simulink model "model"  (R2024b)
settings: Solver=FixedStepDiscrete  StartTime=0.0  StopTime=30  FixedStep=0.1  RelTol=1e-3  EnableMultiTasking=on
libraries: stm32f4xxblockslib x6, stm32g4xxblockslib x2, stm32blockslib x2
(part 2 of 2)

== stateflow chart model/DomoticSystem ==
  state Active_State
    state Config_And_Operations [parallel]
      settings: executionOrder=1
      state Configuration
        state ERROR1
          en:
          uart_transmit_buffer = fromString2Bytes("\r\nInput too long: buffer overflow\r\nPress a key to continue...\r\n")
          uart_out_len = 100;
          ex:
          uart_out_len = 0;
        state Waiting
        state BlindsConfiguration
          state ManageInputBuffer1
            state waitForCompleteInput
              du:
              if uart_in_len == 1
              [input_buffer, new_bf_len, input_ovf] = updateInputBuffer(input_buffer, in_bf_len, uint8(uart_received_char));
              if new_bf_len ~= in_bf_len
              in_bf_len = new_bf_len
              uart_transmit_buffer = printInput(uart_received_char)
              uart_out_len = 1;
              end
              else
              uart_out_len = 0;
              end
              ex:
              uart_out_len = 0;
            (default) -> Active_State.Config_And_Operations.Configuration.BlindsConfiguration.ManageInputBuffer1.waitForCompleteInput
          state Validation
            en:
            [tmp_float_value, success] = asciiBufferToFloat(input_buffer, in_bf_len)
            config_err = ((mod(tmp_float_value, 20) ~= 0) || (tmp_float_value < 0 || tmp_float_value > 180))
          state InitCommunication2
            en:
            input_ovf = false;
            in_bf_len = uint32(0);
            uart_transmit_buffer = reset()
            input_buffer = uart_transmit_buffer(1:20)
            uart_transmit_buffer = cls();
            uart_out_len = 100;
          state PrintLightMenu
            en:
            uart_transmit_buffer = printBlindsMenu()
            uart_out_len = 100;
            ex:
            uart_out_len = 0;
          state SetAngle
            en:
            vblinds_angle = tmp_float_value
            uart_transmit_buffer = fromString2Bytes("\r\nBlinds Configured.\r\nPress a key to continue...\r\n")
            uart_out_len = 100;
            ex:
            uart_out_len = 0;
          state ERROR
            en:
            uart_transmit_buffer = fromString2Bytes("\r\nInvalid Input.\r\nPress a key to continue...\r\n")
            uart_out_len = 100;
            ex:
            uart_out_len = 0;
          state ERROR1
            en:
            uart_transmit_buffer = fromString2Bytes("\r\nInput too long: buffer overflow\r\nPress a key to continue...\r\n")
            uart_out_len = 100;
            ex:
            uart_out_len = 0;
          state Wait
          state Wait1
          state Wait2
          (default) -> Active_State.Config_And_Operations.Configuration.BlindsConfiguration.InitCommunication2
          Active_State.Config_And_Operations.Configuration.BlindsConfiguration.ManageInputBuffer1 -> Active_State.Config_And_Operations.Configuration.BlindsConfiguration.Validation [order 2] : [uart_received_char==EOS && uart_in_len == 1]
          Active_State.Config_And_Operations.Configuration.BlindsConfiguration.PrintLightMenu -> Active_State.Config_And_Operations.Configuration.BlindsConfiguration.ManageInputBuffer1
          Active_State.Config_And_Operations.Configuration.BlindsConfiguration.InitCommunication2 -> Active_State.Config_And_Operations.Configuration.BlindsConfiguration.PrintLightMenu
          Active_State.Config_And_Operations.Configuration.BlindsConfiguration.Validation -> Active_State.Config_And_Operations.Configuration.BlindsConfiguration.ERROR [order 1] : [config_err || ~success]
          Active_State.Config_And_Operations.Configuration.BlindsConfiguration.Validation -> Active_State.Config_And_Operations.Configuration.BlindsConfiguration.SetAngle [order 2]
          Active_State.Config_And_Operations.Configuration.BlindsConfiguration.ManageInputBuffer1 -> Active_State.Config_And_Operations.Configuration.BlindsConfiguration.ERROR1 [order 1] : [input_ovf]
          Active_State.Config_And_Operations.Configuration.BlindsConfiguration.ERROR -> Active_State.Config_And_Operations.Configuration.BlindsConfiguration.Wait
          Active_State.Config_And_Operations.Configuration.BlindsConfiguration.SetAngle -> Active_State.Config_And_Operations.Configuration.BlindsConfiguration.Wait2
          Active_State.Config_And_Operations.Configuration.BlindsConfiguration.ERROR1 -> Active_State.Config_And_Operations.Configuration.BlindsConfiguration.Wait1
          Active_State.Config_And_Operations.Configuration.BlindsConfiguration.Wait -> 466 : [uart_in_len == 1]
          Active_State.Config_And_Operations.Configuration.BlindsConfiguration.Wait1 -> 659 : [uart_in_len == 1]
          Active_State.Config_And_Operations.Configuration.BlindsConfiguration.Wait2 -> BlindsConfiguration : [uart_in_len == 1]{a_config_ended = true;
              | current_config_ended = true;}
        state PrintStatus
          en:
          uart_transmit_buffer = generateConfigurationStatus(isTempValid(temp), isAngleValid(vblinds_angle), isTimeValid(timer), isRelayValid(Relay))
          uart_out_len = 100;
          ex:
          uart_out_len = 0;
        state CheckOldValues
        state ManageInputBuffer
          state waitForCompleteInput
            du:
            if uart_in_len == 1
            [input_buffer, new_bf_len, input_ovf] = updateInputBuffer(input_buffer, in_bf_len, uint8(uart_received_char));
            if new_bf_len ~= in_bf_len
            in_bf_len = new_bf_len
            uart_transmit_buffer = printInput(uart_received_char)
            uart_out_len = 1;
            end
            else
            uart_out_len = 0;
            end
            ex:
            uart_out_len = 0;
          (default) -> Active_State.Config_And_Operations.Configuration.ManageInputBuffer.waitForCompleteInput
        state Validation
          en:
          [tmp_int_value, success] = asciiBufferToInt(input_buffer, in_bf_len)
          config_err = tmp_int_value >  3 || tmp_int_value < 1
        state LightConfiguration
          state InitCommunication3
            en:
            input_ovf = false;
            in_bf_len = uint32(0);
            uart_transmit_buffer = reset()
            input_buffer = uart_transmit_buffer(1:20)
            uart_transmit_buffer = cls();
            uart_out_len = 100;
          state ManageInputBuffer1
            state waitForCompleteInput
              du:
              if uart_in_len == 1
              [input_buffer, new_bf_len, input_ovf] = updateInputBuffer(input_buffer, in_bf_len, uint8(uart_received_char));
              if new_bf_len ~= in_bf_len
              in_bf_len = new_bf_len
              uart_transmit_buffer = printInput(uart_received_char)
              uart_out_len = 1;
              end
              else
              uart_out_len = 0;
              end
              ex:
              uart_out_len = 0;
            (default) -> Active_State.Config_And_Operations.Configuration.LightConfiguration.ManageInputBuffer1.waitForCompleteInput
          state InitCommunication2
            en:
            input_ovf = false;
            in_bf_len = uint32(0);
            uart_transmit_buffer = reset()
            input_buffer = uart_transmit_buffer(1:20)
            uart_transmit_buffer = cls();
            uart_out_len = 100;
          state PrintLightMenu
            en:
            uart_transmit_buffer = printLightMenu1()
            uart_out_len = 100;
            ex:
            uart_out_len = 0;
          state PrintLightTempMenu
            en:
            uart_transmit_buffer = printLightMenu2()
            uart_out_len = 100;
            ex:
            uart_out_len = 0;
          state Validation
            en:
            [tmp_int_value, success] = asciiBufferToInt(input_buffer, in_bf_len)
            config_err = tmp_int_value >  3 || tmp_int_value < 1
          state ManageInputBuffer2
            state waitForCompleteInput
              du:
              if uart_in_len == 1
              [input_buffer, new_bf_len, input_ovf] = updateInputBuffer(input_buffer, in_bf_len, uint8(uart_received_char));
              if new_bf_len ~= in_bf_len
              in_bf_len = new_bf_len
              uart_transmit_buffer = printInput(uart_received_char)
              uart_out_len = 1;
              end
              else
              uart_out_len = 0;
              end
              ex:
              uart_out_len = 0;
            (default) -> Active_State.Config_And_Operations.Configuration.LightConfiguration.ManageInputBuffer2.waitForCompleteInput
          state ERROR1
            en:
            uart_transmit_buffer = fromString2Bytes("\r\nInput too long: buffer overflow\r\nPress a key to continue...\r\n")
            uart_out_len = 100;
            ex:
            uart_out_len = 0;
          state ERROR
            en:
            uart_transmit_buffer = fromString2Bytes("\r\nInvalid Input.\r\nPress a key to continue...\r\n")
            uart_out_len = 100;
            ex:
            uart_out_len = 0;
          state Wait
          state SetLed
            en:
            Relay = boolean(tmp_int_value)
            uart_transmit_buffer = fromString2Bytes("\r\nRelay Configured.\r\nPress a key to continue...\r\n")
            uart_out_len = 100;
            ex:
            uart_out_len = 0;
          state Wait1
          state Validation1
            en:
            [tmp_float_value, success] = asciiBufferToFloat(input_buffer, in_bf_len)
            config_err = ~((tmp_float_value == 0) || (tmp_float_value >= 5 && tmp_float_value <= 30))
          state SetTime
            en:
            timer = tmp_float_value
            uart_transmit_buffer = fromString2Bytes("\r\nTemporization Configured.\r\nPress a key to continue...\r\n")
            uart_out_len = 100;
            ex:
            uart_out_len = 0;
          state Wait2
          Active_State.Config_And_Operations.Configuration.LightConfiguration.Validation -> InitCommunication3 [order 4] : [success && tmp_int_value==3]
          InitCommunication3 -> PrintLightTempMenu
          (default) -> Active_State.Config_And_Operations.Configuration.LightConfiguration.InitCommunication2
          Active_State.Config_And_Operations.Configuration.LightConfiguration.InitCommunication2 -> Active_State.Config_And_Operations.Configuration.LightConfiguration.PrintLightMenu
          Active_State.Config_And_Operations.Configuration.LightConfiguration.PrintLightMenu -> Active_State.Config_And_Operations.Configuration.LightConfiguration.ManageInputBuffer1
          Active_State.Config_And_Operations.Configuration.LightConfiguration.ManageInputBuffer1 -> Active_State.Config_And_Operations.Configuration.LightConfiguration.Validation [order 1] : [uart_received_char==EOS && uart_in_len == 1]
          Active_State.Config_And_Operations.Configuration.LightConfiguration.ManageInputBuffer1 -> Active_State.Config_And_Operations.Configuration.LightConfiguration.ERROR1 [order 2] : [input_ovf]
          PrintLightTempMenu -> ManageInputBuffer2
          Active_State.Config_And_Operations.Configuration.LightConfiguration.Validation -> SetLed [order 2] : [success && tmp_int_value==1]{tmp_int_value=int32(1)}
          Active_State.Config_And_Operations.Configuration.LightConfiguration.Validation -> SetLed [order 3] : [success && tmp_int_value==2]{tmp_int_value=int32(0)}
          Active_State.Config_And_Operations.Configuration.LightConfiguration.Validation -> Active_State.Config_And_Operations.Configuration.LightConfiguration.ERROR [order 1] : [config_err || ~success]
          ManageInputBuffer2 -> Active_State.Config_And_Operations.Configuration.LightConfiguration.ERROR1 [order 2] : [input_ovf]
          Active_State.Config_And_Operations.Configuration.LightConfiguration.ERROR1 -> Active_State.Config_And_Operations.Configuration.LightConfiguration.Wait
          ManageInputBuffer2 -> Validation1 [order 1] : [uart_received_char==EOS && uart_in_len == 1]
          Active_State.Config_And_Operations.Configuration.LightConfiguration.ERROR -> Active_State.Config_And_Operations.Configuration.LightConfiguration.Wait1
          Validation1 -> Active_State.Config_And_Operations.Configuration.LightConfiguration.ERROR [order 1] : [config_err || ~success]
          Active_State.Config_And_Operations.Configuration.LightConfiguration.Wait -> 593 : [uart_in_len == 1]
          Active_State.Config_And_Operations.Configuration.LightConfiguration.Wait1 -> 442 : [uart_in_len == 1]
          SetLed -> Active_State.Config_And_Operations.Configuration.LightConfiguration.Wait2
          Validation1 -> SetTime [order 2] : [success]
          SetTime -> Active_State.Config_And_Operations.Configuration.LightConfiguration.Wait2
          Active_State.Config_And_Operations.Configuration.LightConfiguration.Wait2 -> LightConfiguration : [uart_in_len == 1]{a_config_ended = true;
              | current_config_ended = true;}
        state PrintMenu
          en:
          uart_transmit_buffer=printMenu()
          uart_out_len = 100;
          ex:
          uart_out_len = 0;
        state InitCommunication1
          en:
          input_ovf = false;
          in_bf_len = uint32(0);
          uart_transmit_buffer = reset()
          input_buffer = uart_transmit_buffer(1:20)
          uart_transmit_buffer = cls();
          uart_out_len = 100;
        state init
          en:
          if ~a_config_ended
          a_config_ended  = false
          end
        state feedback
          en:
          uart_transmit_buffer = fromString2Bytes("\r\nInvalid input.\r\nPress a key to continue...\r\n")
          uart_out_len = 100;
          ex:
          uart_out_len = 0;
        state Wait
        state HeatConfiguration
          state ManageInputBuffer1
            state waitForCompleteInput
              du:
              if uart_in_len == 1
              [input_buffer, new_bf_len, input_ovf] = updateInputBuffer(input_buffer, in_bf_len, uint8(uart_received_char));
              if new_bf_len ~= in_bf_len
              in_bf_len = new_bf_len
              uart_transmit_buffer = printInput(uart_received_char)
              uart_out_len = 1;
              end
              else
              uart_out_len = 0;
              end
              ex:
              uart_out_len = 0;
            (default) -> Active_State.Config_And_Operations.Configuration.HeatConfiguration.ManageInputBuffer1.waitForCompleteInput
          state Validation
            en:
            [tmp_float_value, success] = asciiBufferToFloat(input_buffer, in_bf_len)
            config_err = ((abs(mod(tmp_float_value,1)) > 1e-10) || (tmp_float_value < 16 || tmp_float_value > 30))
          state InitCommunication2
            en:
            input_ovf = false;
            in_bf_len = uint32(0);
            uart_transmit_buffer = reset()
            input_buffer = uart_transmit_buffer(1:20)
            uart_transmit_buffer = cls();
            uart_out_len = 100;
          state PrintLightMenu
            en:
            uart_transmit_buffer = printBlindsMenu()
            uart_out_len = 100;
            ex:
            uart_out_len = 0;
          state ERROR
            en:
            uart_transmit_buffer = fromString2Bytes("\r\nInvalid Input.\r\nPress a key to continue...\r\n")
            uart_out_len = 100;
            ex:
            uart_out_len = 0;
          state SetTemp
            en:
            temp = tmp_float_value
            uart_transmit_buffer = fromString2Bytes("\r\nTemperature Configured.\r\nPress a key to continue...\r\n")
            uart_out_len = 100;
            ex:
            uart_out_len = 0;
          state ERROR1
            en:
            uart_transmit_buffer = fromString2Bytes("\r\nInput too long: buffer overflow\r\nPress a key to continue...\r\n")
            uart_out_len = 100;
            ex:
            uart_out_len = 0;
          state Wait1
          state Wait
          state Wait2
          (default) -> Active_State.Config_And_Operations.Configuration.HeatConfiguration.InitCommunication2
          Active_State.Config_And_Operations.Configuration.HeatConfiguration.ManageInputBuffer1 -> Active_State.Config_And_Operations.Configuration.HeatConfiguration.Validation [order 2] : [uart_received_char==EOS && uart_in_len == 1]
          Active_State.Config_And_Operations.Configuration.HeatConfiguration.PrintLightMenu -> Active_State.Config_And_Operations.Configuration.HeatConfiguration.ManageInputBuffer1
          Active_State.Config_And_Operations.Configuration.HeatConfiguration.InitCommunication2 -> Active_State.Config_And_Operations.Configuration.HeatConfiguration.PrintLightMenu
          Active_State.Config_And_Operations.Configuration.HeatConfiguration.Validation -> Active_State.Config_And_Operations.Configuration.HeatConfiguration.ERROR [order 1] : [config_err || ~success]
          Active_State.Config_And_Operations.Configuration.HeatConfiguration.Validation -> SetTemp [order 2]
          Active_State.Config_And_Operations.Configuration.HeatConfiguration.ManageInputBuffer1 -> Active_State.Config_And_Operations.Configuration.HeatConfiguration.ERROR1 [order 1] : [input_ovf]
          Active_State.Config_And_Operations.Configuration.HeatConfiguration.ERROR1 -> Active_State.Config_And_Operations.Configuration.HeatConfiguration.Wait
          Active_State.Config_And_Operations.Configuration.HeatConfiguration.ERROR -> Active_State.Config_And_Operations.Configuration.HeatConfiguration.Wait1
          SetTemp -> Active_State.Config_And_Operations.Configuration.HeatConfiguration.Wait2
          Active_State.Config_And_Operations.Configuration.HeatConfiguration.Wait -> 601 : [uart_in_len == 1]
          Active_State.Config_And_Operations.Configuration.HeatConfiguration.Wait1 -> 482 : [uart_in_len == 1]
          Active_State.Config_And_Operations.Configuration.HeatConfiguration.Wait2 -> HeatConfiguration : [uart_in_len == 1]{a_config_ended = true;
              | current_config_ended = true;}
        CheckOldValues -> init
        Waiting -> CheckOldValues : [uart_in_len == 1]
        Active_State.Config_And_Operations.Configuration.ERROR1 -> Waiting
        ManageInputBuffer -> Active_State.Config_And_Operations.Configuration.ERROR1 [order 2] : [input_ovf]
        BlindsConfiguration -> Configuration : [current_config_ended]
        Active_State.Config_And_Operations.Configuration.Validation -> BlindsConfiguration [order 1] : [tmp_int_value == 1]{current_config_ended=false}
        660 -> CheckOldValues
        473 -> CheckOldValues
        602 -> CheckOldValues
        596 -> CheckOldValues
        480 -> CheckOldValues
        443 -> CheckOldValues
        PrintStatus -> PrintMenu
        PrintMenu -> ManageInputBuffer
        Active_State.Config_And_Operations.Configuration.Validation -> LightConfiguration [order 3] : [tmp_int_value == 2]{current_config_ended=false}
        ManageInputBuffer -> Active_State.Config_And_Operations.Configuration.Validation [order 1] : [uart_received_char==EOS && uart_in_len == 1]
        LightConfiguration -> Configuration : [current_config_ended]
        Active_State.Config_And_Operations.Configuration.Validation -> HeatConfiguration [order 4] : [tmp_int_value == 3]{current_config_ended=false}
        InitCommunication1 -> PrintStatus
        init -> InitCommunication1
        Active_State.Config_And_Operations.Configuration.Validation -> feedback [order 2] : [~success || config_err]
        Active_State.Config_And_Operations.Configuration.Wait -> InitCommunication1 : [uart_in_len == 1]
        (default) -> init
        feedback -> Active_State.Config_And_Operations.Configuration.Wait
        HeatConfiguration -> Configuration : [current_config_ended]
      state WaitForRelease1
      state Operational
        state HeatingManagement [parallel]
          settings: executionOrder=4
          state range_1
            en:
            Heating_R = 255;
            Heating_G = 255;
            Heating_B = 0;
          state range_2
            en:
            Heating_R = 128;
            Heating_G = 255;
            Heating_B = 128;
          state range_4
            en:
            Heating_R = 0;
            Heating_G = 128;
            Heating_B = 255;
          state range_3
            en:
            Heating_R = 0;
            Heating_G = 0;
            Heating_B = 255;
          state range_5
            en:
            Heating_R = 0;
            Heating_G = 255;
            Heating_B = 255;
          (default) -> (junction 715)
          range_5 -> (junction 715) : [temp>30]
          (junction 715) -> range_1 [order 1] : [temp>=16 && temp<=18]
          (junction 715) -> range_5 [order 5] : [temp>= 28 && temp<=30]
          range_1 -> (junction 715) : [temp>18]
          range_4 -> (junction 715) : [temp>27]
          (junction 715) -> range_2 [order 2] : [temp>=19 && temp<=21]
          (junction 715) -> range_4 [order 4] : [temp>= 25 && temp<=27]
          range_2 -> (junction 715) : [temp>21]
          range_3 -> (junction 715) : [temp>24]
          (junction 715) -> range_3 [order 3] : [temp>=22 && temp<=24]
        state LightManagement [parallel]
          settings: executionOrder=2
          state Relay
            state Operation
              state OFF
                state WaitForButtonPressing
                state Debounce
                state Turn_off
                  en:
                  Relay=OFF;
                Active_State.Config_And_Operations.Operational.LightManagement.Relay.Operation.OFF.Debounce -> Active_State.Config_And_Operations.Operational.LightManagement.Relay.Operation.OFF.WaitForButtonPressing : after(debounce, sec)
                Turn_off -> Active_State.Config_And_Operations.Operational.LightManagement.Relay.Operation.OFF.Debounce : [button_light_pressed==OFF]
                (default) -> Turn_off
              state ON
                state Turn_ON
                  en:
                  Relay=ON
                state Debounce
                state WaitForButtonPressing
                (default) -> Turn_ON
                Turn_ON -> Active_State.Config_And_Operations.Operational.LightManagement.Relay.Operation.ON.Debounce : [button_light_pressed==OFF]
                Active_State.Config_And_Operations.Operational.LightManagement.Relay.Operation.ON.Debounce -> Active_State.Config_And_Operations.Operational.LightManagement.Relay.Operation.ON.WaitForButtonPressing : after(debounce, sec)
              (default) -> (junction 643)
              (junction 643) -> Active_State.Config_And_Operations.Operational.LightManagement.Relay.Operation.ON [order 2] : [Relay==ON]
              (junction 643) -> Active_State.Config_And_Operations.Operational.LightManagement.Relay.Operation.OFF [order 1] : [Relay==OFF]
              Active_State.Config_And_Operations.Operational.LightManagement.Relay.Operation.OFF.WaitForButtonPressing -> Active_State.Config_And_Operations.Operational.LightManagement.Relay.Operation.ON : [button_light_pressed==ON]
              Active_State.Config_And_Operations.Operational.LightManagement.Relay.Operation.ON.WaitForButtonPressing -> Turn_off : [button_light_pressed==ON]
            state Debounce
            state Temp
              state GoToRelay [parallel]
                settings: executionOrder=1
                state WaitForPressing
                (default) -> WaitForPressing
              state EllapsedTime [parallel]
                settings: executionOrder=2
                state Wait
                  en:
                  Relay=ON;
                (default) -> Active_State.Config_And_Operations.Operational.LightManagement.Relay.Temp.EllapsedTime.Wait
            state WaitForRelease
            state Debounce1
            (default) -> Operation
            Active_State.Config_And_Operations.Operational.LightManagement.Relay.Temp.EllapsedTime.Wait -> Operation : [after(timer, sec)]{Relay=OFF}
            Active_State.Config_And_Operations.Operational.LightManagement.Relay.Debounce -> Operation : after(debounce, sec){Relay=OFF}
            Operation -> Active_State.Config_And_Operations.Operational.LightManagement.Relay.WaitForRelease : [button_temp_pressed==ON && uint32(timer) ~= 0]
            WaitForPressing -> Active_State.Config_And_Operations.Operational.LightManagement.Relay.Debounce : [button_light_pressed==ON && button_temp_pressed==OFF]
            Active_State.Config_And_Operations.Operational.LightManagement.Relay.WaitForRelease -> Active_State.Config_And_Operations.Operational.LightManagement.Relay.Debounce1 : [button_temp_pressed==OFF]
            Active_State.Config_And_Operations.Operational.LightManagement.Relay.Debounce1 -> Temp : [after(debounce, sec)]
          (default) -> Relay
        state NotifyUART [parallel]
          settings: executionOrder=3
          state Invia
            en:
            uart_transmit_buffer = messageForUART(Relay,vblinds_angle,temp,timer)
            uart_out_len = 100
            ex:
            uart_out_len = 0
          state Wait
          (default) -> Invia
          Invia -> Active_State.Config_And_Operations.Operational.NotifyUART.Wait
          Active_State.Config_And_Operations.Operational.NotifyUART.Wait -> Invia : after(10, sec)
        state VBlindsManagement [parallel]
          settings: executionOrder=1
          state SetAngle
            du:
            servo_pwm_out = 5.0 + (vblinds_angle / 180.0) * 20.0;
          (default) -> Active_State.Config_And_Operations.Operational.VBlindsManagement.SetAngle
      state Debounce3
      state WaitForRelease
      state Debounce2
      (junction 674) -> Configuration [order 1] : [first_config]
      (default) -> (junction 674)
      (junction 674) -> Operational [order 2]
      Configuration -> WaitForRelease1 : [a_config_ended  == true && button_config_pressed==ON && isTempValid(temp) && isAngleValid(vblinds_angle) && isTimeValid(timer) && isRelayValid(Relay)]{first_config=false}
      WaitForRelease1 -> Debounce3 : [button_temp_pressed==OFF]
      Debounce3 -> Operational : after(debounce, sec)
      Active_State.Config_And_Operations.WaitForRelease -> Debounce2 : [button_temp_pressed==OFF]
      Debounce2 -> Configuration : after(debounce, sec){a_config_ended = false}
      Operational -> Active_State.Config_And_Operations.WaitForRelease : [button_config_pressed==ON]
    state BlinkingManagement [parallel]
      settings: executionOrder=2
      state ON
        en:
        Blinking=ON
      state OFF
        en:
        Blinking=OFF
      (default) -> Active_State.BlinkingManagement.ON
      Active_State.BlinkingManagement.OFF -> Active_State.BlinkingManagement.ON : after(1/(2*blinking_hz), sec)
      Active_State.BlinkingManagement.ON -> Active_State.BlinkingManagement.OFF : after(1/(2*blinking_hz), sec)
  state PopValues
    en:
    tmp_float_value = tmp_float_value_Old_Session;
    Relay = Relay_Old_Session;
    Heating_R = Heating_R_Old_Session ;
    Heating_G = Heating_G_Old_Session;
    Heating_B = Heating_B_Old_Session;
    servo_pwm_out = servo_pwm_out_Old_Session;
    vblinds_angle = vblinds_angle_Old_Session;
  state Debounce
    en:
    uart_out_len = 0
  state WaitForRelese
    en:
    uart_transmit_buffer = cls()
    uart_out_len = 100
    ex:
    uart_out_len = 0
  state OFF_STATE
    en:
    % Push Values
    Relay_Old_Session = Relay;
    Heating_R_Old_Session = Heating_R;
    Heating_G_Old_Session = Heating_G;
    Heating_B_Old_Session = Heating_B;
    servo_pwm_out_Old_Session = servo_pwm_out;
    vblinds_angle_Old_Session = vblinds_angle;
    tmp_float_value_Old_Session = tmp_float_value
    % Tutto Spento
    Blinking=OFF;
    Relay = OFF;
    Heating_R = 255;
    Heating_G = 255;
    Heating_B = 255;
    servo_pwm_out = 5.0;
    vblinds_angle = 0.0;
    %Print
    uart_transmit_buffer = fromString2Bytes(sprintf('\033[0;0H\033[2J') + "[Inactive State]");
    uart_out_len = 100;
    ex:
    uart_out_len = 0;
  state Wait
  state WaitForRelese1
    en:
    uart_transmit_buffer = cls()
    uart_out_len = 100
    ex:
    uart_out_len = 0
  state Debounce1
    en:
    uart_out_len = 0
  PopValues -> Active_State
  Debounce -> PopValues : after(debounce, sec)
  WaitForRelese -> Debounce : [power_button_pressed==OFF]
  (default) -> OFF_STATE
  Wait -> WaitForRelese : [power_button_pressed==ON]
  OFF_STATE -> Wait
  Active_State -> WaitForRelese1 : [power_button_pressed==ON]
  WaitForRelese1 -> Debounce1 : [power_button_pressed==OFF]
  Debounce1 -> OFF_STATE : after(debounce, sec)
  data: buffer function_output uint8 size=100; buffer function_output uint8 size=100; buffer function_output uint8 size=100; buffer function_output uint8 size=100; isTempValid function_input; isAngleValid function_input; isTimeValid function_input; isRelayValid function_input; msg function_output; msg_len function_output; input_buffer function_input uint8 size=20; length function_input uint32 size=1; inputChar function_input uint8 size=1; new_input_buffer function_output uint8 size=20; newLength function_output uint32 size=1; overflow function_output boolean size=1; buffer function_output uint8 size=100; buffer function_input; length function_input; value function_output; success function_output; buffer function_output uint8 size=100; input function_input uint8 size=1; buffer function_input; length function_input; value function_output; success function_output; input_buffer function_input; formatted_buffer function_output; out_len function_output; buffer function_output uint8 size=100; angle function_input; validation function_output; temp function_input; validation function_output; relay function_input boolean size=1; validation function_output boolean size=1; str function_input; msg function_output; time function_input; validation function_output; buffer function_output uint8 size=100; relay function_input boolean size=1; angle function_input; temperature function_input double size=1; temporization function_input double size=1; msg function_output uint8 size=100; msg_len function_output uint32 size=1; ON constant boolean =1; OFF constant boolean =0; Relay output boolean size=1 =0; button_light_pressed input boolean size=1; button_temp_pressed input boolean size=1; debounce local double size=1 =0.05; timer local double size=1 =-1; blinking_hz local double size=1 =2; Blinking output; Heating_B output uint8 size=1 =255; Heating_R output uint8 size=1 =255; Heating_G output uint8 size=1 =255; button_config_pressed input boolean size=1; uart_transmit_buffer output uint8 size=100; uart_out_len output uint8 size=1; uart_received_char input uint8 size=1; uart_in_len input uint32 size=1; input_buffer local uint8 size=20; in_bf_len local uint32 size=1; EOS constant uint8 =13; tmp_int_value local int32 size=1 =0; success local boolean size=1 =0; tmp_float_value local double size=1 =-1.0; config_err local boolean size=1 =0; new_bf_len local uint32 size=1; vblinds_angle local double size=1 =-1; temp local double size=1 =-1; input_ovf local boolean size=1; current_config_ended local; a_config_ended local boolean size=1 =0; power_button_pressed input boolean size=1; servo_pwm_out output double size=1; first_config local boolean size=1 =true; Heating_B_Old_Session local; Heating_G_Old_Session local; Heating_R_Old_Session local; Relay_Old_Session local; servo_pwm_out_Old_Session local; vblinds_angle_Old_Session local; tmp_float_value_Old_Session local
  function buffer = printBlindsMenu:
    | function buffer = printBlindsMenu() %#codegen
    | % Restituisce un vettore uint8 (MAX_LEN × 1) con il menu testuale.
    | 
    | MAX_LEN = 100;
    | buffer  = zeros(MAX_LEN, 1, 'uint8');
    | idx     = int32(1);
    | 
    | % Char-matrix a lunghezza fissa (ogni riga 25 caratteri in questo esempio)
    | menu = [ ...
    |     'Blinds Menu:                                          '; ... % 
    |     'Insert the angle in degree with a resolution of 20    '; ... % 
    |     'inclusive range: 0-180                                '
    |     'Insert:                                               '  ... %
    | ];
    | 
    | nLines  = size(menu, 1);
    | nCols   = size(menu, 2);            % lunghezza fissa di ogni riga
    | 
    | for i = 1:nLines
    |     % Trova l’ultima colonna non-spazio della riga i
    |     last = int32(0);
    |     for c = nCols:-1:1
    |         if menu(i, c) ~= ' '
    |             last = int32(c);
    |             break;
    |         end
    |     end
    | 
    |     % Copia i caratteri utili
    |     for k = int32(1):last
    |         buffer(idx) = uint8(menu(i, k));
    |         idx = idx + 1;
    |     end
    |     
    |     % tmp = buffer(1:199)
    |     % Aggiunge newline '\n'
    |     buffer(idx) = uint8(10);
    |     idx = idx + 1;
    |     buffer(idx) = uint8(13);
    |     idx = idx + 1;
    | end
    | end
  function buffer = printLightMenu1:
    | function buffer = printLightMenu1() %#codegen
    | % Restituisce un vettore uint8 (MAX_LEN × 1) con il menu testuale.
    | 
    | MAX_LEN = 100;
    | buffer  = zeros(MAX_LEN, 1, 'uint8');
    | idx     = int32(1);
    | 
    | % Char-matrix a lunghezza fissa (ogni riga 25 caratteri in questo esempio)
    | menu = [ ...
    |     'Light Menu:      '; ... % 
    |     '1 - Turn On      '; ... % 
    |     '2 - Turn Off     '; ... % 
    |     '3 - Temporization'; ... % 
    |     'Insert:          '  ... %
    | ];
    | 
    | nLines  = size(menu, 1);
    | nCols   = size(menu, 2);            % lunghezza fissa di ogni riga
    | 
    | for i = 1:nLines
    |     % Trova l’ultima colonna non-spazio della riga i
    |     last = int32(0);
    |     for c = nCols:-1:1
    |         if menu(i, c) ~= ' '
    |             last = int32(c);
    |             break;
    |         end
    |     end
    | 
    |     % Copia i caratteri utili
    |     for k = int32(1):last
    |         buffer(idx) = uint8(menu(i, k));
    |         idx = idx + 1;
    |     end
    |     
    |     % tmp = buffer(1:199)
    |     % Aggiunge newline '\n'
    |     buffer(idx) = uint8(10);
    |     idx = idx + 1;
    |     buffer(idx) = uint8(13);
    |     idx = idx + 1;
    | end
    | end
  function buffer = printLightMenu2:
    | function buffer = printLightMenu2() %#codegen
    | % Restituisce un vettore uint8 (MAX_LEN × 1) con il menu testuale.
    | 
    | MAX_LEN = 100;
    | buffer  = zeros(MAX_LEN, 1, 'uint8');
    | idx     = int32(1);
    | 
    | % Char-matrix a lunghezza fissa (ogni riga 25 caratteri in questo esempio)
    | menu = [ ...
    |     'Temporization Menu:                                                    '; ... % 
    |     'You can either enter 0 or a value between the inclusive range 5...30   '; ... % 
    |     'Insert:                                                                '  ... %
    | ];
    | 
    | nLines  = size(menu, 1);
    | nCols   = size(menu, 2);            % lunghezza fissa di ogni riga
    | 
    | for i = 1:nLines
    |     % Trova l’ultima colonna non-spazio della riga i
    |     last = int32(0);
    |     for c = nCols:-1:1
    |         if menu(i, c) ~= ' '
    |             last = int32(c);
    |             break;
    |         end
    |     end
    | 
    |     % Copia i caratteri utili
    |     for k = int32(1):last
    |         buffer(idx) = uint8(menu(i, k));
    |         idx = idx + 1;
    |     end
    |     
    |     % tmp = buffer(1:199)
    |     % Aggiunge newline '\n'
    |     buffer(idx) = uint8(10);
    |     idx = idx + 1;
    |     buffer(idx) = uint8(13);
    |     idx = idx + 1;
    | end
    | end
  function buffer = printBlindsMenu:
    | function buffer = printBlindsMenu() %#codegen
    | % Restituisce un vettore uint8 (MAX_LEN × 1) con il menu testuale.
    | 
    | MAX_LEN = 100;
    | buffer  = zeros(MAX_LEN, 1, 'uint8');
    | idx     = int32(1);
    | 
    | % Char-matrix a lunghezza fissa (ogni riga 25 caratteri in questo esempio)
    | menu = [ ...
    |     'Heating Menu:                    '; ... % 
    |     'Insert the temperature in celsius'; ... %
    |     'Resolution: 1 C                  '
    |     'Inclusive range: 16-30           '
    |     'Insert:                          '  ... %
    | ];
    | 
    | nLines  = size(menu, 1);
    | nCols   = size(menu, 2);            % lunghezza fissa di ogni riga
    | 
    | for i = 1:nLines
    |     % Trova l’ultima colonna non-spazio della riga i
    |     last = int32(0);
    |     for c = nCols:-1:1
    |         if menu(i, c) ~= ' '
    |             last = int32(c);
    |             break;
    |         end
    |     end
    | 
    |     % Copia i caratteri utili
    |     for k = int32(1):last
    |         buffer(idx) = uint8(menu(i, k));
    |         idx = idx + 1;
    |     end
    |     
    |     % tmp = buffer(1:199)
    |     % Aggiunge newline '\n'
    |     buffer(idx) = uint8(10);
    |     idx = idx + 1;
    |     buffer(idx) = uint8(13);
    |     idx = idx + 1;
    | end
    | end
  function [msg, msg_len] = generateConfigurationStatus(isTempValid, isAngleValid, isTimeValid, isRelayValid):
    | function [msg, msg_len] = generateConfigurationStatus(isTempValid, isAngleValid, isTimeValid, isRelayValid)
    | %#codegen
    | % Questa funzione genera la linea di stato per il menu di configurazione.
    | % Es: 
    | % [Configuration]
    | % Tempe: x Angle: o Timer: x Relay: o
    | % È progettata per essere efficiente e compatibile con Stateflow (#codegen).
    | 
    |     % Buffer per contenere il messaggio. 128 è più che sufficiente.
    |     MAX_LEN = 100;
    |     persistent msg_buffer
    |     if isempty(msg_buffer)
    |         msg_buffer = zeros(MAX_LEN, 1, 'uint8');
    |     end
    |     
    |     % Pulisce il buffer per ogni nuova chiamata.
    |     msg_buffer(:) = 0;
    |     
    |     % Usa uint32 per il contatore per compatibilità con l'output msg_len.
    |     idx = uint32(1);
    |     
    |     % --- Costruzione del Messaggio ---
    | 
    |     % Riga 1: Titolo e a capo
    |     [msg_buffer, idx] = write_string('[Configuration]', msg_buffer, idx);
    |     msg_buffer(idx) = uint8(10); % Newline (LF, \n)
    |     idx = idx + 1;
    |     msg_buffer(idx) = uint8(13); % Carriage Return (LF, \r)
    |     idx = idx + 1;
    |     
    |     % Riga 2: Stato delle variabili
    |     
    |     % Temperatura
    |     [msg_buffer, idx] = write_string('Tempe: ', msg_buffer, idx);
    |     if isTempValid
    |         msg_buffer(idx) = uint8('o');
    |     else
    |         msg_buffer(idx) = uint8('x');
    |     end
    |     idx = idx + 1;
    |     
    |     % Angolo (con spazio iniziale per separare)
    |     [msg_buffer, idx] = write_string(' Angle: ', msg_buffer, idx);
    |     if isAngleValid
    |         msg_buffer(idx) = uint8('o');
    |     else
    |         msg_buffer(idx) = uint8('x');
    |     end
    |     idx = idx + 1;
    | 
    |     % Timer (con spazio iniziale)
    |     [msg_buffer, idx] = write_string(' Timer: ', msg_buffer, idx);
    |     if isTimeValid
    |         msg_buffer(idx) = uint8('o');
    |     else
    |         msg_buffer(idx) = uint8('x');
    |     end
    |     idx = idx + 1;
    | 
    |     % Relay (con spazio iniziale)
    |     [msg_buffer, idx] = write_string(' Relay: ', msg_buffer, idx);
    |     if isRelayValid
    |         msg_buffer(idx) = uint8('o');
    |     else
    |         msg_buffer(idx) = uint8('x');
    |     end
    |     idx = idx + 1;
    | 
    |     % --- Terminazione del messaggio completo (LF + CR) ---
    |     msg_buffer(idx) = uint8(10); % LF (\n)
    |     idx = idx + 1;
    |     msg_buffer(idx) = uint8(13); % CR (\r)
    |     idx = idx + 1;
    |     
    |     % Imposta i valori di output
    |     msg_len = idx - 1;
    |     msg = msg_buffer;
    | end
    | 
    | 
    | % --- FUNZIONE LOCALE DI SUPPORTO ---
    | 
    | function [msg, idx_out] = write_string(str, msg, idx_in)
    | %#codegen
    | % Scrive una stringa di caratteri nel buffer in modo efficiente.
    |     str_as_uint8 = uint8(str);
    |     len = uint32(numel(str_as_uint8)); % Usa uint32 per coerenza
    |     for k = 1:len
    |         % L'indice del buffer deve essere un intero, quindi usiamo (idx_in + k - 1)
    |         % e Coder gestisce la conversione da uint32 a double per l'indicizzazione.
    |         msg(idx_in + (k - 1)) = str_as_uint8(k);
    |     end
    |     idx_out = idx_in + len;
    | end
  function [new_input_buffer, newLength, overflow] = updateInputBuffer(input_buffer, length, inputChar):
    | function [new_input_buffer, newLength, overflow] = updateInputBuffer(input_buffer, length, inputChar)
    | %#codegen
    | % Aggiorna un buffer di input con un nuovo carattere.
    | % Gestisce cifre, backspace e invio (che termina la stringa con '\0').
    | 
    | MAX_LEN = 20;
    | overflow = false;
    | new_input_buffer = input_buffer;
    | newLength = length;
    | inputChar = uint8((inputChar));
    | 
    | % Se il carattere è una cifra '0'-'9'
    | if inputChar >= uint8(('0')) && inputChar <= uint8(('9'))
    |     if newLength < MAX_LEN
    |         new_input_buffer(newLength + 1) = inputChar;
    |         newLength = newLength + 1;
    |     else
    |         overflow = true;
    |     end
    | 
    | % Se il carattere è BACKSPACE (ASCII 8) o DELETE (ASCII 127)
    | elseif inputChar == 8 || inputChar == 127
    |     if newLength > 0
    |         % Rimuove l'ultimo carattere (non è necessario azzerarlo se
    |         % la lunghezza è gestita correttamente, ma è una buona pratica)
    |         new_input_buffer(newLength) = uint8((0)); 
    |         newLength = newLength - 1;
    |     end
    | 
    | % Se il carattere è INVIO (ENTER, ASCII 13)
    | elseif inputChar == 13
    |     % Aggiunge il terminatore di stringa C-style '\0'
    |     if newLength < MAX_LEN
    |         new_input_buffer(newLength + 1) = uint8((0));
    |         % Non è necessario incrementare newLength per il terminatore,
    |         % perché la lunghezza utile non lo include. Ma se lo fai,
    |         % assicurati di essere coerente. Lasciamolo così per ora.
    |     else
    |         overflow = true;
    |     end
    |     % La logica che riempie il resto del buffer con zeri è superflua
    |     % se la funzione di conversione si ferma al primo zero, ma la manteniamo
    |     % per sicurezza e pulizia del buffer.
    |     for k = newLength+2:MAX_LEN
    |         new_input_buffer(k) = uint8((0));
    |     end
    | elseif inputChar == uint8(('.'))
    |     already_used = false;
    |     for i=1:newLength
    |         if new_input_buffer(i) == uint8(('.'))
    |             already_used = true;
    |             break
    |         end
    |     end
    |     if already_used == false
    |         if newLength + 1 < MAX_LEN
    |             new_input_buffer(newLength + 1) = inputChar;
    |             newLength = newLength + 1;
    |         else
    |             overflow = true;
    |         end
    |     end
    | else
    |     % Ignora esplicitamente tutti gli altri caratteri.
    |     % Se 'inputChar' è un carattere non gestito (es. 'a', '!', o un codice
    |     % di escape inviato dal tasto CANC), la funzione non farà nulla,
    |     % restituendo il buffer e la lunghezza inalterati.
    |     % Questo risolve il tuo problema.
    | end
    | 
    | 
    | 
    | return
    | end
  function buffer = printMenu:
    | function buffer = printMenu() %#codegen
    | % Restituisce un vettore uint8 (MAX_LEN × 1) con il menu testuale.
    | 
    | MAX_LEN = 100;
    | buffer  = zeros(MAX_LEN, 1, 'uint8');
    | idx     = int32(1);
    | 
    | % Char-matrix a lunghezza fissa (ogni riga 25 caratteri in questo esempio)
    | menu = [ ...
    |     'Config Menu:            '; ... % 
    |     '1 - Blinds Configuration'; ... % 
    |     '2 - Light Configuration '; ... % 
    |     '3 - Heat Configuration  '; ... % 
    |     'Insert:                 '  ... %
    | ];
    | 
    | nLines  = size(menu, 1);
    | nCols   = size(menu, 2);            % lunghezza fissa di ogni riga
    | 
    | for i = 1:nLines
    |     % Trova l’ultima colonna non-spazio della riga i
    |     last = int32(0);
    |     for c = nCols:-1:1
    |         if menu(i, c) ~= ' '
    |             last = int32(c);
    |             break;
    |         end
    |     end
    | 
    |     % Copia i caratteri utili
    |     for k = int32(1):last
    |         buffer(idx) = uint8(menu(i, k));
    |         idx = idx + 1;
    |     end
    |     
    |     % tmp = buffer(1:199)
    |     % Aggiunge newline '\n'
    |     buffer(idx) = uint8(10);
    |     idx = idx + 1;
    |     buffer(idx) = uint8(13);
    |     idx = idx + 1;
    | end
    | end
  function [value, success] = asciiBufferToInt(buffer, length):
    | function [value, success] = asciiBufferToInt(buffer, length)
    | %#codegen
    | % Converte un buffer di caratteri ASCII in un intero a 32 bit.
    | % Si ferma al primo carattere nullo '\0' o alla fine della 'length' data.
    | 
    | value = int32(0);
    | success = true;
    | 
    | if length == 0
    |     success = false;
    |     return;
    | end
    | 
    | sign = int32(1);
    | startIdx = 1;
    | 
    | % Gestisce il segno
    | if buffer(1) == uint8('-')
    |     sign = int32(-1);
    |     startIdx = 2;
    | elseif buffer(1) == uint8('+')
    |     startIdx = 2;
    | end
    | 
    | % Itera sui caratteri fino alla lunghezza specificata
    | for i = startIdx:length
    |     c = buffer(i);
    |     
    |     % Se incontra il terminatore di stringa, la conversione è finita e ha successo
    |     if c == 0
    |         break;
    |     end
    |     
    |     % Se il carattere non è una cifra, la conversione fallisce
    |     if c < '0' || c > '9'
    |         success = false;
    |         value = int32(0); % Resetta il valore in caso di fallimento
    |         return;
    |     end
    |     
    |     % Aggiorna il valore
    |     digit = int32(c - uint8('0'));
    |     value = value * 10 + digit;
    | end
    | 
    | value = value * sign;
    | end
  function buffer = printInput(input):
    | function buffer = printInput(input)%#codegen
    | 
    | MAX_LEN = 100;
    | buffer  = zeros(MAX_LEN, 1, 'uint8');
    | 
    | 
    | % Aggiunge newline '\n'
    | buffer(1) = input;
    | 
    | end
  function [value, success] = asciiBufferToFloat(buffer, length):
    | function [value, success] = asciiBufferToFloat(buffer, length)
    | %#codegen
    | value = 0.0;
    | success = true;
    | sign = 1.0;
    | i = 1;
    | hasDecimal = false;
    | decimalFactor = 0.1;
    | 
    | if length == 0
    |     success = false;
    |     return;
    | end
    | 
    | if buffer(i) == uint8('-')
    |     sign = -1.0;
    |     i = i + 1;
    | elseif buffer(i) == uint8('+')
    |     i = i + 1;
    | end
    | 
    | while i <= length
    |     c = buffer(i);
    |     if c == 0  % terminatore \0
    |         break;
    |     end
    |     if c == uint8('.') && ~hasDecimal
    |         hasDecimal = true;
    |         i = i + 1;
    |         continue;
    |     elseif c >= uint8('0') && c <= uint8('9')
    |         digit = double(c - uint8('0'));
    |         if ~hasDecimal
    |             value = value * 10.0 + digit;
    |         else
    |             value = value + digit * decimalFactor;
    |             decimalFactor = decimalFactor * 0.1;
    |         end
    |     else
    |         success = false;
    |         return;
    |     end
    |     i = i + 1;
    | end
    | 
    | value = value * sign;
    | end
  function [formatted_buffer, out_len] = formatBufferToFixedString(input_buffer):
    | function [formatted_buffer, out_len] = formatBufferToFixedString(input_buffer)
    | %#codegen
    | % Questa funzione prende un buffer di codici ASCII e li converte in una stringa
    | % leggibile. I caratteri stampabili vengono mostrati come tali, quelli non
    | % stampabili vengono mostrati come <valore numerico>.
    | 
    |     formatted_buffer = zeros(100, 1, 'uint8');
    |     out_len = 0;
    |     current_pos = 1;
    |     lookup_table = uint8('0123456789'); % Per stampare i valori numerici
    | 
    |     formatted_buffer(current_pos) = uint8('['); current_pos = current_pos + 1;
    | 
    |     for i = 1:20
    |         c = input_buffer(i);
    | 
    |         % Controlla se il carattere è stampabile (da ' ' a '~')
    |         if c >= 32 && c <= 126
    |             % È stampabile, mostralo tra apici
    |             formatted_buffer(current_pos) = uint8(''''); current_pos = current_pos + 1;
    |             formatted_buffer(current_pos) = c;       current_pos = current_pos + 1;
    |             formatted_buffer(current_pos) = uint8(''''); current_pos = current_pos + 1;
    |         else
    |             % NON è stampabile, mostra il suo valore numerico tra < >
    |             formatted_buffer(current_pos) = uint8('<'); current_pos = current_pos + 1;
    |             
    |             % --- Usa la nostra logica di conversione numero->stringa ---
    |             c1=uint8(0); c2=uint8(0); c3=uint8(0); str_len=0;
    |             if c > 99
    |                 c1 = lookup_table(floor(c / 100) + 1);
    |                 c2 = lookup_table(mod(floor(c / 10), 10) + 1);
    |                 c3 = lookup_table(mod(c, 10) + 1);
    |                 str_len = 3;
    |             elseif c > 9
    |                 c1 = lookup_table(floor(c / 10) + 1);
    |                 c2 = lookup_table(mod(c, 10) + 1);
    |                 str_len = 2;
    |             else
    |                 c1 = lookup_table(c + 1);
    |                 str_len = 1;
    |             end
    |             if str_len == 3
    |                 formatted_buffer(current_pos) = c1; current_pos=current_pos+1;
    |                 formatted_buffer(current_pos) = c2; current_pos=current_pos+1;
    |                 formatted_buffer(current_pos) = c3; current_pos=current_pos+1;
    |             elseif str_len == 2
    |                 formatted_buffer(current_pos) = c1; current_pos=current_pos+1;
    |                 formatted_buffer(current_pos) = c2; current_pos=current_pos+1;
    |             else
    |                 formatted_buffer(current_pos) = c1; current_pos=current_pos+1;
    |             end
    |             % --- Fine logica conversione ---
    |             
    |             formatted_buffer(current_pos) = uint8('>'); current_pos = current_pos + 1;
    |         end
    | 
    |         if i < 20
    |             formatted_buffer(current_pos) = uint8(','); current_pos = current_pos + 1;
    |             formatted_buffer(current_pos) = uint8(' '); current_pos = current_pos + 1;
    |         end
    |     end
    | 
    |     formatted_buffer(current_pos) = uint8(']'); current_pos = current_pos + 1;
    |     out_len = current_pos - 1;
    | end
  function buffer = cls:
    | function buffer = cls() %#codegen
    |     MAX_LEN  = 100;
    |     buffer   = zeros(MAX_LEN,1,'uint8');
    | 
    |     % char vector, not string scalar
    |     clsString = sprintf('\033[0;0H\033[2J');
    | 
    |     for k = 1:numel(clsString)
    |         buffer(k) = uint8(clsString(k));   % clsString(k) is one char
    |     end
    | end
  function validation = isAngleValid(angle):
    | function validation = isAngleValid(angle)
    | validation = (mod(angle, 20) == 0 && (angle>=0 && angle<=180));
    | return 
    | end
  function validation = isTempValid(temp):
    | function validation = isTempValid(temp)
    | validation =  ((abs(mod(temp,1)) < 1e-10) && (temp >= 16 && temp <= 30));
    | return 
    | end
  function validation = isRelayValid(relay):
    | function validation = isRelayValid(relay)
    | validation = relay == 0 || relay == 1;
    | return
    | end
  function msg = fromString2Bytes(str):
    | function msg = fromString2Bytes(str)
    | %#codegen
    | 
    | MAX_LEN = 100;
    | msg = zeros(MAX_LEN, 1, 'uint8');
    | 
    | % Trasforma in char se necessario
    | str = char(str);
    | 
    | % Converti sequenze escape
    | str = replace(str, '\n', char(10));   % newline
    | str = replace(str, '\r', char(13));   % carriage return
    | str = replace(str, '\t', char(9));    % tab
    | 
    | n = min(length(str), MAX_LEN);
    | for i = 1:n
    |     msg(i) = uint8(str(i));
    | end
    | 
    | % Il resto del buffer rimane a 0 (padding)
    | end
  function validation = isTimeValid(time):
    | function validation = isTimeValid(time)
    | validation = (time== 0 || (time>=5 && time<=30));
    | return 
    | end
  function buffer = reset:
    | function buffer = reset() %#codegen
    | 
    | MAX_LEN = 100;
    | buffer  = zeros(MAX_LEN, 1, 'uint8');
    | 
    | end
  function [msg, msg_len] = messageForUART(relay, angle, temperature, temporization):
    | function [msg, msg_len] = messageForUART(relay, angle, temperature, temporization)
    | %#codegen
    | % Versione modificata per generare un messaggio di stato operativo.
    | % VERSIONE CORRETTA 2: Risolve l'errore di type-mismatch per msg_len,
    | % cambiando il tipo del contatore 'idx' in uint32.
    | 
    |     MAX_LEN = 100;
    |     persistent msg_buffer
    |     if isempty(msg_buffer)
    |         msg_buffer = zeros(MAX_LEN, 1, 'uint8');
    |     end
    |     
    |     msg_buffer(:) = 0;
    |     
    |     % --- CORREZIONE CHIAVE QUI ---
    |     % Inizializza 'idx' come uint32 per farlo corrispondere al tipo di output 'msg_len'.
    |     idx = uint32(1); 
    | 
    |     % --- Composizione del messaggio ---
    |     
    |     msg_buffer = cls();
    |     idx = uint32(11);
    | 
    |     [msg_buffer, idx] = write_string('[Operational]', msg_buffer, idx);
    |     msg_buffer(idx) = uint8(10); % LF (\n)
    |     idx = idx + 1;
    |     msg_buffer(idx) = uint8(13); % LF (\r)
    |     idx = idx + 1;
    | 
    |     [msg_buffer, idx] = write_string('Relay=', msg_buffer, idx);
    |     if relay
    |         msg_buffer(idx) = uint8('1');
    |     else
    |         msg_buffer(idx) = uint8('0');
    |     end
    |     idx = idx + 1;
    |     [msg_buffer, idx] = write_string(',', msg_buffer, idx);
    | 
    |     [msg_buffer, idx] = write_string('Angle=', msg_buffer, idx);
    |     [msg_buffer, idx] = write_float_decimal(angle, 1, msg_buffer, idx);
    |     [msg_buffer, idx] = write_string(',', msg_buffer, idx);
    | 
    |     [msg_buffer, idx] = write_string('Temperature=', msg_buffer, idx);
    |     [msg_buffer, idx] = write_float_decimal(temperature, 1, msg_buffer, idx);
    |     [msg_buffer, idx] = write_string(',', msg_buffer, idx);
    | 
    |     [msg_buffer, idx] = write_string('Temporization=', msg_buffer, idx);
    |     [msg_buffer, idx] = write_float_decimal(temporization, 1, msg_buffer, idx);
    | 
    |     % --- Terminazione del messaggio ---
    |     msg_buffer(idx) = uint8(10); % LF (\n)
    |     idx = idx + 1;
    |     msg_buffer(idx) = uint8(13); % CR (\r)
    |     idx = idx + 1;
    |     
    |     % Ora il tipo di (idx - 1) è uint32, che corrisponde a msg_len
    |     msg_len = idx - 1;
    |     msg = msg_buffer;
    | end
    | 
    | 
    | % --- FUNZIONI LOCALI DI SUPPORTO ---
    | 
    | function [msg, idx_out] = write_string(str, msg, idx_in)
    | %#codegen
    |     str_as_uint8 = uint8(str);
    |     len = numel(str_as_uint8);
    |     for k = 1:len
    |         msg(idx_in + uint32(k - 1)) = str_as_uint8(k);
    |     end
    |     idx_out = idx_in + uint32(len);
    | end
    | 
    | function [msg, idx_out] = write_float_decimal(val, num_decimals, msg, idx_in)
    | %#codegen
    |     idx = idx_in;
    |     
    |     is_negative = val < 0;
    |     if is_negative
    |         msg(idx) = uint8('-');
    |         idx = idx + 1;
    |         val = -val;
    |     end
    | 
    |     scale = 10^num_decimals;
    |     int_part = uint32(floor(val));
    |     frac_part = uint32(round(mod(val, 1) * scale));
    | 
    |     [msg, idx] = write_uint_decimal(int_part, msg, idx);
    |     
    |     msg(idx) = uint8('.');
    |     idx = idx + 1;
    |     
    |     [msg, idx] = write_uint_decimal(frac_part, msg, idx);
    |     
    |     idx_out = idx;
    | end
    | 
    | 
    | function [msg, idx_out] = write_uint_decimal(val, msg, idx_in)
    | %#codegen
    |     persistent lut;
    |     if isempty(lut)
    |         lut = uint8('0123456789');
    |     end
    |     
    |     idx = idx_in;
    | 
    |     if val > 999
    |         val = uint32(999); 
    |     end
    | 
    |     if val > 99
    |         h = idivide(val, uint32(100), 'floor');
    |         t = idivide(mod(val, 100), uint32(10), 'floor');
    |         u = mod(val, 10);
    |         
    |         msg(idx)     = lut(h + 1);
    |         msg(idx + 1) = lut(t + 1);
    |         msg(idx + 2) = lut(u + 1);
    |         idx = idx + 3;
    |         
    |     elseif val > 9
    |         t = idivide(val, uint32(10), 'floor');
    |         u = mod(val, 10);
    |         
    |         msg(idx)     = lut(t + 1);
    |         msg(idx + 1) = lut(u + 1);
    |         idx = idx + 2;
    |         
    |     else
    |         msg(idx) = lut(val + 1);
    |         idx = idx + 1;
    |     end
    |     
    |     idx_out = idx;
    | end
